simulink model "s_b4a4x1kf"  (R2018a)
settings: Solver=VariableStepDiscrete  StartTime=0.0  StopTime=1  RelTol=1e-3
undefined symbols (not defined in the file): fft_stages, n_bits_ants, n_bits_xengs
libraries: xbsIndex_r4 x22055, xbsReplacements_r4 x30, casper_library_misc x29, casper_library_scopes x15, xps_library x4
(part 72 of 227)

== system s_b4a4x1kf/sys1/vacc_tvg0/ins_vector ==
  new_acc_in : Inport
  data_in : Inport  Port=2
  valid_in : Inport  Port=3
  vector : Inport  Port=4
  value : Inport  Port=5
  enable : Inport  Port=6
  misci : Inport  Port=7
  Delay : xbsIndex_r4/Delay  rst=off  infoeditControl=Selection of Reset will increase slice count due to use of real FFs and instead of SRLs  en=off  latency=2  reg_retiming=off  dbl_ovrd=off  block_type=delay
      settings: xl_area=[0, 0, 0, 0, 0, 0, 0]
  Delay1 : xbsIndex_r4/Delay  rst=off  infoeditControl=Selection of Reset will increase slice count due to use of real FFs and instead of SRLs  en=off  latency=2  reg_retiming=off  dbl_ovrd=off  block_type=delay
      settings: xl_area=[0, 0, 0, 0, 0, 0, 0]
  Delay2 : xbsIndex_r4/Delay  rst=off  infoeditControl=Selection of Reset will increase slice count due to use of real FFs and instead of SRLs  en=off  latency=2  reg_retiming=off  dbl_ovrd=off  block_type=delay
      settings: xl_area=[0, 0, 0, 0, 0, 0, 0]
  Delay3 : xbsIndex_r4/Delay  rst=off  infoeditControl=Selection of Reset will increase slice count due to use of real FFs and instead of SRLs  en=off  latency=3  reg_retiming=on  dbl_ovrd=off  block_type=delay
      settings: xl_area=[0, 0, 0, 0, 0, 0, 0]
  Delay4 : xbsIndex_r4/Delay  rst=off  infoeditControl=Selection of Reset will increase slice count due to use of real FFs and instead of SRLs  en=off  latency=1  reg_retiming=on  dbl_ovrd=off  block_type=delay
      settings: xl_area=[0, 0, 0, 0, 0, 0, 0]
  Delay5 : xbsIndex_r4/Delay  rst=off  infoeditControl=Selection of Reset will increase slice count due to use of real FFs and instead of SRLs  en=off  latency=3  reg_retiming=on  dbl_ovrd=off  block_type=delay
      settings: xl_area=[0, 0, 0, 0, 0, 0, 0]
  Gateway Out{1..6} (6 alike) : xbsIndex_r4/Gateway Out  inherit_from_input=off  hdl_port=off  rows=1  columns=1  UseAsDAC=off  DACChannel='1'  interface=None  automatic_assignment=on  address_offset=hex2dec('00')  intf_name=''  intf_description=''  timing_constraint=None  locs_specified=off  LOCs={}  io_standard={}  block_type=gatewayout
      settings: infoedit="Gateway out block.  Converts Xilinx fixed point inputs into ouputs of type Simulink integer, double, or fixed point.<P><P>Hardware notes:  In hardware these blocks become top level output ports or are discarded, depending on how they are configured."  xl_area=[0, 0, 0, 0, 0, 0, 0]  block_version=10.1.3
  Logical : xbsIndex_r4/Logical  logical_function=AND  inputs=2  en=off  latency=0  precision=Full  arith_type=Unsigned  n_bits=8  bin_pt=2  align_bp=on  dbl_ovrd=off  block_type=logical
      settings: xl_area=[0, 0, 0, 0, 0, 0, 0]
  Mux : xbsIndex_r4/Mux  inputs=2  en=off  latency=1  precision=Full  arith_type="Signed  (2's comp)"  n_bits=8  bin_pt=2  quantization=Truncate  overflow=Wrap  dbl_ovrd=off  block_type=mux
      settings: xl_area=[0, 0, 0, 0, 0, 0, 0]
  Relational : xbsIndex_r4/Relational  mode=a=b  op_type=Bool  en=off  latency=1  dbl_ovrd=off  block_type=relational
      settings: xl_area=[0, 0, 0, 0, 0, 0, 0]  block_version=10.1.3
  Scope2 : Scope  NumInputPorts=6
  tot_cntr : xbsIndex_r4/Counter  cnt_type=Count Limited  cnt_to=num_vectors-1  operation=Up  start_count=0  cnt_by_val=1  arith_type=Unsigned  n_bits=ceil(log2(num_vectors-1))  bin_pt=0  load_pin=off  rst=on  en=on  explicit_period=on  period=1  use_behavioral_HDL=off  implementation=Fabric  use_rpm=on  dbl_ovrd=off  block_type=counter
      settings: xl_area=[0, 0, 0, 0, 0, 0, 0]
  new_acc_out : Outport
  data : Outport  Port=2
  valid_out : Outport  Port=3
  misco : Outport  Port=4
  wires:
  enable/1 -> Logical/1
  Gateway Out5/1 -> Scope2/3
  Gateway Out4/1 -> Scope2/2
  Gateway Out6/1 -> Scope2/1
  Gateway Out1/1 -> Scope2/4
  valid_in/1 -> Delay4/1
  Mux/1 -> data/1, Gateway Out6/1
  tot_cntr/1 -> Gateway Out2/1, Relational/1
  vector/1 -> Relational/2
  data_in/1 -> Delay1/1
  value/1 -> Delay2/1
  Delay/1 -> valid_out/1, Gateway Out4/1
  Logical/1 -> Mux/1, Gateway Out3/1
  Relational/1 -> Logical/2
  Gateway Out2/1 -> Scope2/5
  Delay1/1 -> Mux/2
  Delay3/1 -> new_acc_out/1
  new_acc_in/1 -> Delay3/1, tot_cntr/1, Gateway Out1/1
  Delay4/1 -> tot_cntr/2, Delay/1, Gateway Out5/1
  Delay2/1 -> Mux/3
  Gateway Out3/1 -> Scope2/6
  misci/1 -> Delay5/1
  Delay5/1 -> misco/1

== system s_b4a4x1kf/sys1/vacc_tvg0/n_per_group ==
  sim_1 : Inport
  convert1_1 : DataTypeConversion  OutDataTypeStr=fixdt('ufix32_En0')  LockScale=on
  convert2_1 : DataTypeConversion  OutDataTypeStr=fixdt('ufix32_En0')  ConvertRealWorld=Stored Integer (SI)  LockScale=on
  gain_1 : Gain
  io_delay : xbsIndex_r4/Delay  rst=off  infoeditControl=Selection of Reset will increase slice count due to use of real FFs and instead of SRLs  en=off  latency=0  reg_retiming=on  dbl_ovrd=off  block_type=delay
  reint1 : xbsIndex_r4/Reinterpret  force_arith_type=on  arith_type=Unsigned  force_bin_pt=on  bin_pt=0  block_type=reinterpret
  s_b4a4x1kf_sys1_vacc_tvg0_n_per_group_user_data_out : xbsIndex_r4/Gateway In  gui_display_data_type=Fixed-point  arith_type=Unsigned  n_bits=32  bin_pt=0  preci_type=Single  exp_width=8  frac_width=24  rows=1  columns=1  quantization="Round  (unbiased: +/- Inf)"  overflow=Saturate  period=1  UseAsADC=off  ADCChannel='1'  interface=None  automatic_assignment=on  address_offset=hex2dec('00')  intf_name=''  intf_description=''  default_value=0  timing_constraint=None  locs_specified=off  LOCs={}  io_standard={}  inherit_from_input=off  hdl_port=on  dbl_ovrd=off  block_type=gatewayin
  slice_reg : xbsIndex_r4/Slice  nbits=32  boolean_output=off  mode=Lower Bit Location + Width  bit1=0  base1=MSB of Input  bit0=0  base0=LSB of Input  dbl_ovrd=off  block_type=slice
  in_reg : Outport
  wires:
  s_b4a4x1kf_sys1_vacc_tvg0_n_per_group_user_data_out/1 -> io_delay/1
  sim_1/1 -> convert1_1/1
  convert1_1/1 -> convert2_1/1
  convert2_1/1 -> gain_1/1
  gain_1/1 -> s_b4a4x1kf_sys1_vacc_tvg0_n_per_group_user_data_out/1
  io_delay/1 -> slice_reg/1
  slice_reg/1 -> reint1/1
  reint1/1 -> in_reg/1

== system s_b4a4x1kf/sys1/vacc_tvg0/n_pulses ==
  sim_1 : Inport
  convert1_1 : DataTypeConversion  OutDataTypeStr=fixdt('ufix32_En0')  LockScale=on
  convert2_1 : DataTypeConversion  OutDataTypeStr=fixdt('ufix32_En0')  ConvertRealWorld=Stored Integer (SI)  LockScale=on
  gain_1 : Gain
  io_delay : xbsIndex_r4/Delay  rst=off  infoeditControl=Selection of Reset will increase slice count due to use of real FFs and instead of SRLs  en=off  latency=0  reg_retiming=on  dbl_ovrd=off  block_type=delay
  reint1 : xbsIndex_r4/Reinterpret  force_arith_type=on  arith_type=Unsigned  force_bin_pt=on  bin_pt=0  block_type=reinterpret
  s_b4a4x1kf_sys1_vacc_tvg0_n_pulses_user_data_out : xbsIndex_r4/Gateway In  gui_display_data_type=Fixed-point  arith_type=Unsigned  n_bits=32  bin_pt=0  preci_type=Single  exp_width=8  frac_width=24  rows=1  columns=1  quantization="Round  (unbiased: +/- Inf)"  overflow=Saturate  period=1  UseAsADC=off  ADCChannel='1'  interface=None  automatic_assignment=on  address_offset=hex2dec('00')  intf_name=''  intf_description=''  default_value=0  timing_constraint=None  locs_specified=off  LOCs={}  io_standard={}  inherit_from_input=off  hdl_port=on  dbl_ovrd=off  block_type=gatewayin
  slice_reg : xbsIndex_r4/Slice  nbits=32  boolean_output=off  mode=Lower Bit Location + Width  bit1=0  base1=MSB of Input  bit0=0  base0=LSB of Input  dbl_ovrd=off  block_type=slice
  in_reg : Outport
  wires:
  s_b4a4x1kf_sys1_vacc_tvg0_n_pulses_user_data_out/1 -> io_delay/1
  sim_1/1 -> convert1_1/1
  convert1_1/1 -> convert2_1/1
  convert2_1/1 -> gain_1/1
  gain_1/1 -> s_b4a4x1kf_sys1_vacc_tvg0_n_pulses_user_data_out/1
  io_delay/1 -> slice_reg/1
  slice_reg/1 -> reint1/1
  reint1/1 -> in_reg/1

== system s_b4a4x1kf/sys1/vacc_tvg0/pipeline1 ==
  d : Inport
  Register0 : xbsIndex_r4/Register  init=0  rst=off  en=off  dbl_ovrd=off  block_type=register
      settings: block_version=11.4
  Register1 : xbsIndex_r4/Register  init=0  rst=off  en=off  dbl_ovrd=off  block_type=register
      settings: block_version=11.4
  Register2 : xbsIndex_r4/Register  init=0  rst=off  en=off  dbl_ovrd=off  block_type=register
      settings: block_version=11.4
  q : Outport
  wires:
  Register0/1 -> Register1/1
  Register1/1 -> Register2/1
  d/1 -> Register0/1
  Register2/1 -> q/1

== system s_b4a4x1kf/sys1/vacc_tvg0/pipeline2 ==
  d : Inport
  Register0 : xbsIndex_r4/Register  init=0  rst=off  en=off  dbl_ovrd=off  block_type=register
      settings: block_version=11.4
  Register1 : xbsIndex_r4/Register  init=0  rst=off  en=off  dbl_ovrd=off  block_type=register
      settings: block_version=11.4
  Register2 : xbsIndex_r4/Register  init=0  rst=off  en=off  dbl_ovrd=off  block_type=register
      settings: block_version=11.4
  q : Outport
  wires:
  Register0/1 -> Register1/1
  Register1/1 -> Register2/1
  d/1 -> Register0/1
  Register2/1 -> q/1

== system s_b4a4x1kf/sys1/vacc_tvg0/pipeline3 ==
  d : Inport
  Register0 : xbsIndex_r4/Register  init=0  rst=off  en=off  dbl_ovrd=off  block_type=register
      settings: block_version=11.4
  Register1 : xbsIndex_r4/Register  init=0  rst=off  en=off  dbl_ovrd=off  block_type=register
      settings: block_version=11.4
  Register2 : xbsIndex_r4/Register  init=0  rst=off  en=off  dbl_ovrd=off  block_type=register
      settings: block_version=11.4
  q : Outport
  wires:
  Register0/1 -> Register1/1
  Register1/1 -> Register2/1
  d/1 -> Register0/1
  Register2/1 -> q/1

== system s_b4a4x1kf/sys1/vacc_tvg0/pipeline4 ==
  d : Inport
  Register0 : xbsIndex_r4/Register  init=0  rst=off  en=off  dbl_ovrd=off  block_type=register
      settings: block_version=11.4
  Register1 : xbsIndex_r4/Register  init=0  rst=off  en=off  dbl_ovrd=off  block_type=register
      settings: block_version=11.4
  Register2 : xbsIndex_r4/Register  init=0  rst=off  en=off  dbl_ovrd=off  block_type=register
      settings: block_version=11.4
  q : Outport
  wires:
  Register0/1 -> Register1/1
  Register1/1 -> Register2/1
  d/1 -> Register0/1
  Register2/1 -> q/1

== system s_b4a4x1kf/sys1/vacc_tvg0/pipeline7 ==
  d : Inport
  Register0 : xbsIndex_r4/Register  init=0  rst=off  en=off  dbl_ovrd=off  block_type=register
      settings: block_version=11.4
  Register1 : xbsIndex_r4/Register  init=0  rst=off  en=off  dbl_ovrd=off  block_type=register
      settings: block_version=11.4
  Register2 : xbsIndex_r4/Register  init=0  rst=off  en=off  dbl_ovrd=off  block_type=register
      settings: block_version=11.4
  q : Outport
  wires:
  Register0/1 -> Register1/1
  Register1/1 -> Register2/1
  d/1 -> Register0/1
  Register2/1 -> q/1

== system s_b4a4x1kf/sys1/vacc_tvg0/ts_offset ==
  sim_1 : Inport
  convert1_1 : DataTypeConversion  OutDataTypeStr=fixdt('ufix32_En0')  LockScale=on
  convert2_1 : DataTypeConversion  OutDataTypeStr=fixdt('ufix32_En0')  ConvertRealWorld=Stored Integer (SI)  LockScale=on
  gain_1 : Gain
  io_delay : xbsIndex_r4/Delay  rst=off  infoeditControl=Selection of Reset will increase slice count due to use of real FFs and instead of SRLs  en=off  latency=0  reg_retiming=on  dbl_ovrd=off  block_type=delay
  reint1 : xbsIndex_r4/Reinterpret  force_arith_type=on  arith_type=Unsigned  force_bin_pt=on  bin_pt=0  block_type=reinterpret
  s_b4a4x1kf_sys1_vacc_tvg0_ts_offset_user_data_out : xbsIndex_r4/Gateway In  gui_display_data_type=Fixed-point  arith_type=Unsigned  n_bits=32  bin_pt=0  preci_type=Single  exp_width=8  frac_width=24  rows=1  columns=1  quantization="Round  (unbiased: +/- Inf)"  overflow=Saturate  period=1  UseAsADC=off  ADCChannel='1'  interface=None  automatic_assignment=on  address_offset=hex2dec('00')  intf_name=''  intf_description=''  default_value=0  timing_constraint=None  locs_specified=off  LOCs={}  io_standard={}  inherit_from_input=off  hdl_port=on  dbl_ovrd=off  block_type=gatewayin
  slice_reg : xbsIndex_r4/Slice  nbits=32  boolean_output=off  mode=Lower Bit Location + Width  bit1=0  base1=MSB of Input  bit0=0  base0=LSB of Input  dbl_ovrd=off  block_type=slice
  in_reg : Outport
  wires:
  s_b4a4x1kf_sys1_vacc_tvg0_ts_offset_user_data_out/1 -> io_delay/1
  sim_1/1 -> convert1_1/1
  convert1_1/1 -> convert2_1/1
  convert2_1/1 -> gain_1/1
  gain_1/1 -> s_b4a4x1kf_sys1_vacc_tvg0_ts_offset_user_data_out/1
  io_delay/1 -> slice_reg/1
  slice_reg/1 -> reint1/1
  reint1/1 -> in_reg/1

== system s_b4a4x1kf/sys1/vacc_tvg0/write ==
  sim_1 : Inport
  convert1_1 : DataTypeConversion  OutDataTypeStr=fixdt('ufix32_En0')  LockScale=on
  convert2_1 : DataTypeConversion  OutDataTypeStr=fixdt('ufix32_En0')  ConvertRealWorld=Stored Integer (SI)  LockScale=on
  gain_1 : Gain
  io_delay : xbsIndex_r4/Delay  rst=off  infoeditControl=Selection of Reset will increase slice count due to use of real FFs and instead of SRLs  en=off  latency=0  reg_retiming=on  dbl_ovrd=off  block_type=delay
  reint1 : xbsIndex_r4/Reinterpret  force_arith_type=on  arith_type=Unsigned  force_bin_pt=on  bin_pt=0  block_type=reinterpret
  s_b4a4x1kf_sys1_vacc_tvg0_write_user_data_out : xbsIndex_r4/Gateway In  gui_display_data_type=Fixed-point  arith_type=Unsigned  n_bits=32  bin_pt=0  preci_type=Single  exp_width=8  frac_width=24  rows=1  columns=1  quantization="Round  (unbiased: +/- Inf)"  overflow=Saturate  period=1  UseAsADC=off  ADCChannel='1'  interface=None  automatic_assignment=on  address_offset=hex2dec('00')  intf_name=''  intf_description=''  default_value=0  timing_constraint=None  locs_specified=off  LOCs={}  io_standard={}  inherit_from_input=off  hdl_port=on  dbl_ovrd=off  block_type=gatewayin
  slice_reg : xbsIndex_r4/Slice  nbits=32  boolean_output=off  mode=Lower Bit Location + Width  bit1=0  base1=MSB of Input  bit0=0  base0=LSB of Input  dbl_ovrd=off  block_type=slice
  in_reg : Outport
  wires:
  s_b4a4x1kf_sys1_vacc_tvg0_write_user_data_out/1 -> io_delay/1
  sim_1/1 -> convert1_1/1
  convert1_1/1 -> convert2_1/1
  convert2_1/1 -> gain_1/1
  gain_1/1 -> s_b4a4x1kf_sys1_vacc_tvg0_write_user_data_out/1
  io_delay/1 -> slice_reg/1
  slice_reg/1 -> reint1/1
  reint1/1 -> in_reg/1

== system s_b4a4x1kf/sys1/xeng/auto_tap ==
  a_del : Inport
  a_ndel : Inport  Port=2
  a_loop : Inport  Port=3
  acc_in : Inport  Port=4
  valid_in : Inport  Port=5
  sync_in : Inport  Port=6
  delay : Subsystem  mask(delay_bram){DelayLen=510, bram_latency=7, use_dsp48=off, async=off}
      mask prompts: DelayLen "Delay By:"; bram_latency "BRAM Latency"; use_dsp48 "Use DSP48"; async "asynchronous operation"
      mask help: A delay block that uses BRAM for its storage.
      mask init:
      | delay_bram_init(gcb, ...
      |     'DelayLen', DelayLen, ...
      |     'bram_latency', bram_latency, ...
      |     'use_dsp48', use_dsp48, ...
      |     'async', async);
      mask Help: eval('xlWeb(''http://casper.berkeley.edu/wiki/Delay_bram'')')
  dual_pol_cmac : Subsystem  mask{acc_len=256, n_bits_in=8, bin_pt_in=7, mult_latency=4, add_latency=3, multiplier_implementation=embedded multiplier core}
      mask prompts: acc_len "Number of accumulations"; n_bits_in "Number of bits in"; bin_pt_in "Binary point in"; mult_latency "Multiplier latency"; add_latency "Adder latency"; multiplier_implementation "Multiplier implementation"
      mask init: same as s_b4a4x1kf/sys0/xeng/auto_tap/dual_pol_cmac
      mask TypeOptions multiplier_implementation: behavioral HDL | standard core | embedded multiplier core
  sync_delay : Subsystem  mask(sync_delay){DelayLen=267}
      mask prompts: DelayLen "Delay Length:"
      mask help: Delay an infrequent boolean pulse by the specified number of clocks.
      mask init:
      | BitWidth = max(2, ceil(log2(DelayLen+1)));
      | UseCounter = 1;
      | if DelayLen == 0,
      | 	UseCounter = 0;
      | end
      mask Help: eval('xlWeb(''http://casper.berkeley.edu/wiki/Sync_delay'')')
      mask Display: fprintf('Z^-%d', DelayLen)
  a_del_out : Outport
  a_ndel_out : Outport  Port=2
  a_end_out : Outport  Port=3
  acc_out : Outport  Port=4
  valid_out : Outport  Port=5
  rst_out : Outport  Port=6
  sync_out : Outport  Port=7
  wires:
  sync_delay/1(Out) -> sync_out/1
  delay/1(dout) -> a_end_out/1
  a_loop/1 -> delay/1(din)
  a_ndel/1 -> a_ndel_out/1, dual_pol_cmac/2(a2)
  valid_in/1 -> dual_pol_cmac/5(valid_in)
  dual_pol_cmac/2(valid_out) -> valid_out/1
  acc_in/1 -> dual_pol_cmac/3(acc_in)
  dual_pol_cmac/1(acc_out) -> acc_out/1
  a_del/1 -> a_del_out/1, dual_pol_cmac/1(a1)
  sync_in/1 -> rst_out/1, dual_pol_cmac/4(sync), sync_delay/1(In)

== system s_b4a4x1kf/sys1/xeng/baseline_tap1 ==
  a_del : Inport
  a_ndel : Inport  Port=2
  a_end : Inport  Port=3
  acc_in : Inport  Port=4
  valid_in : Inport  Port=5
  rst : Inport  Port=6
  sync1 : Inport  Port=7
  Constant : xbsIndex_r4/Constant  const=ant_sep * acc_len  gui_display_data_type=Fixed-point  arith_type=Unsigned  n_bits=ant_bits + bit_growth  bin_pt=0  preci_type=Single  exp_width=8  frac_width=24  explicit_period=on  period=1  equ=P=C  opselect=C  inp2=PCIN>>17  opr=+  inp1=P  carry=CIN  dbl_ovrd=off  block_type=constant
      settings: block_version=9.1.01
  Convert : xbsIndex_r4/Convert  gui_display_data_type=Fixed-point  arith_type=Unsigned  n_bits=1  bin_pt=0  float_type=Single  exp_bits=8  fraction_bits=24  quantization=Truncate  overflow=Wrap  en=off  latency=0  pipeline=off  dbl_ovrd=off  block_type=convert
      settings: xl_area=[0, 0, 0, 0, 0, 0, 0]
  Counter : xbsIndex_r4/Counter  cnt_type=Count Limited  cnt_to=n_ants * acc_len - 1  operation=Up  start_count=0  cnt_by_val=1  arith_type=Unsigned  n_bits=ant_bits + bit_growth  bin_pt=0  load_pin=off  rst=on  en=off  explicit_period=off  period=1  use_behavioral_HDL=off  implementation=Fabric  use_rpm=on  dbl_ovrd=off  block_type=counter
      settings: xl_area=[0, 0, 0, 0, 0, 0, 0]  block_version=9.1.01
  Delay{1,3,7..8} (4 alike) : xbsIndex_r4/Delay  rst=off  infoeditControl=Selection of Reset will increase slice count due to use of real FFs and instead of SRLs  en=off  latency=1  reg_retiming=on  dbl_ovrd=off  block_type=delay
      settings: xl_area=[0, 0, 0, 0, 0, 0, 0]  block_version=9.1.01
  Mux : xbsIndex_r4/Mux  inputs=2  en=off  latency=1  precision=Full  arith_type="Signed  (2's comp)"  n_bits=8  bin_pt=2  quantization=Truncate  overflow=Wrap  dbl_ovrd=off  block_type=mux
      settings: xl_area=[0, 0, 0, 0, 0, 0, 0]  block_version=9.1.01
  Relational : xbsIndex_r4/Relational  mode=a<b  op_type=Bool  en=off  latency=0  dbl_ovrd=off  block_type=relational
      settings: xl_area=[0, 0, 0, 0, 0, 0, 0]  block_version=9.1.01
  delay : Subsystem  mask(delay_bram){DelayLen=acc_len, bram_latency=bram_latency, use_dsp48=off, async=off}
      mask prompts: DelayLen "Delay By:"; bram_latency "BRAM Latency"; use_dsp48 "Use DSP48"; async "asynchronous operation"
      mask help: A delay block that uses BRAM for its storage.
      mask init:
      | delay_bram_init(gcb, ...
      |     'DelayLen', DelayLen, ...
      |     'bram_latency', bram_latency, ...
      |     'use_dsp48', use_dsp48, ...
      |     'async', async);
      mask Help: eval('xlWeb(''http://casper.berkeley.edu/wiki/Delay_bram'')')
  dual_pol_cmac : Subsystem  mask{acc_len=256, n_bits_in=8, bin_pt_in=7, mult_latency=4, add_latency=3, multiplier_implementation=embedded multiplier core}
      mask prompts: acc_len "Number of accumulations"; n_bits_in "Number of bits in"; bin_pt_in "Binary point in"; mult_latency "Multiplier latency"; add_latency "Adder latency"; multiplier_implementation "Multiplier implementation"
      mask init: same as s_b4a4x1kf/sys0/xeng/auto_tap/dual_pol_cmac
      mask TypeOptions multiplier_implementation: behavioral HDL | standard core | embedded multiplier core
  a_del_out : Outport
  a_ndel_out : Outport  Port=2
  a_end_out : Outport  Port=3
  acc_out : Outport  Port=4
  valid_out : Outport  Port=5
  rst_out : Outport  Port=6
  sync_out : Outport  Port=7
  wires:
  delay/1(dout) -> Delay3/1
  Mux/1 -> dual_pol_cmac/2(a2)
  Counter/1 -> Relational/1
  Constant/1 -> Relational/2
  Relational/1 -> Convert/1
  Convert/1 -> Mux/1
  rst/1 -> Delay1/1, Counter/1
  a_del/1 -> delay/1(din)
  dual_pol_cmac/1(acc_out) -> acc_out/1
  acc_in/1 -> dual_pol_cmac/3(acc_in)
  dual_pol_cmac/2(valid_out) -> valid_out/1
  valid_in/1 -> dual_pol_cmac/5(valid_in)
  a_ndel/1 -> Mux/2, Delay7/1
  a_end/1 -> Mux/3, Delay8/1
  Delay3/1 -> a_del_out/1, dual_pol_cmac/1(a1)
  Delay7/1 -> a_ndel_out/1
  Delay8/1 -> a_end_out/1
  Delay1/1 -> rst_out/1, dual_pol_cmac/4(sync)
  sync1/1 -> sync_out/1

== system s_b4a4x1kf/sys1/xeng/baseline_tap2 ==
  a_del : Inport
  a_ndel : Inport  Port=2
  a_end : Inport  Port=3
  acc_in : Inport  Port=4
  valid_in : Inport  Port=5
  rst : Inport  Port=6
  sync1 : Inport  Port=7
  Constant : xbsIndex_r4/Constant  const=ant_sep * acc_len  gui_display_data_type=Fixed-point  arith_type=Unsigned  n_bits=ant_bits + bit_growth  bin_pt=0  preci_type=Single  exp_width=8  frac_width=24  explicit_period=on  period=1  equ=P=C  opselect=C  inp2=PCIN>>17  opr=+  inp1=P  carry=CIN  dbl_ovrd=off  block_type=constant
      settings: block_version=9.1.01
  Convert : xbsIndex_r4/Convert  gui_display_data_type=Fixed-point  arith_type=Unsigned  n_bits=1  bin_pt=0  float_type=Single  exp_bits=8  fraction_bits=24  quantization=Truncate  overflow=Wrap  en=off  latency=0  pipeline=off  dbl_ovrd=off  block_type=convert
      settings: xl_area=[0, 0, 0, 0, 0, 0, 0]
  Counter : xbsIndex_r4/Counter  cnt_type=Count Limited  cnt_to=n_ants * acc_len - 1  operation=Up  start_count=0  cnt_by_val=1  arith_type=Unsigned  n_bits=ant_bits + bit_growth  bin_pt=0  load_pin=off  rst=on  en=off  explicit_period=off  period=1  use_behavioral_HDL=off  implementation=Fabric  use_rpm=on  dbl_ovrd=off  block_type=counter
      settings: xl_area=[0, 0, 0, 0, 0, 0, 0]  block_version=9.1.01
  Delay{1,3,7..8} (4 alike) : xbsIndex_r4/Delay  rst=off  infoeditControl=Selection of Reset will increase slice count due to use of real FFs and instead of SRLs  en=off  latency=1  reg_retiming=on  dbl_ovrd=off  block_type=delay
      settings: xl_area=[0, 0, 0, 0, 0, 0, 0]  block_version=9.1.01
  Mux : xbsIndex_r4/Mux  inputs=2  en=off  latency=1  precision=Full  arith_type="Signed  (2's comp)"  n_bits=8  bin_pt=2  quantization=Truncate  overflow=Wrap  dbl_ovrd=off  block_type=mux
      settings: xl_area=[0, 0, 0, 0, 0, 0, 0]  block_version=9.1.01
  Relational : xbsIndex_r4/Relational  mode=a<b  op_type=Bool  en=off  latency=0  dbl_ovrd=off  block_type=relational
      settings: xl_area=[0, 0, 0, 0, 0, 0, 0]  block_version=9.1.01
  delay : Subsystem  mask(delay_bram){DelayLen=acc_len, bram_latency=bram_latency, use_dsp48=off, async=off}
      mask prompts: DelayLen "Delay By:"; bram_latency "BRAM Latency"; use_dsp48 "Use DSP48"; async "asynchronous operation"
      mask help: A delay block that uses BRAM for its storage.
      mask init:
      | delay_bram_init(gcb, ...
      |     'DelayLen', DelayLen, ...
      |     'bram_latency', bram_latency, ...
      |     'use_dsp48', use_dsp48, ...
      |     'async', async);
      mask Help: eval('xlWeb(''http://casper.berkeley.edu/wiki/Delay_bram'')')
  dual_pol_cmac : Subsystem  mask{acc_len=256, n_bits_in=8, bin_pt_in=7, mult_latency=4, add_latency=3, multiplier_implementation=embedded multiplier core}
      mask prompts: acc_len "Number of accumulations"; n_bits_in "Number of bits in"; bin_pt_in "Binary point in"; mult_latency "Multiplier latency"; add_latency "Adder latency"; multiplier_implementation "Multiplier implementation"
      mask init: same as s_b4a4x1kf/sys0/xeng/auto_tap/dual_pol_cmac
      mask TypeOptions multiplier_implementation: behavioral HDL | standard core | embedded multiplier core
  a_del_out : Outport
  a_ndel_out : Outport  Port=2
  a_end_out : Outport  Port=3
  acc_out : Outport  Port=4
  valid_out : Outport  Port=5
  rst_out : Outport  Port=6
  sync_out : Outport  Port=7
  wires:
  delay/1(dout) -> Delay3/1
  Mux/1 -> dual_pol_cmac/2(a2)
  Counter/1 -> Relational/1
  Constant/1 -> Relational/2
  Relational/1 -> Convert/1
  Convert/1 -> Mux/1
  rst/1 -> Delay1/1, Counter/1
  a_del/1 -> delay/1(din)
  dual_pol_cmac/1(acc_out) -> acc_out/1
  acc_in/1 -> dual_pol_cmac/3(acc_in)
  dual_pol_cmac/2(valid_out) -> valid_out/1
  valid_in/1 -> dual_pol_cmac/5(valid_in)
  a_ndel/1 -> Mux/2, Delay7/1
  a_end/1 -> Mux/3, Delay8/1
  Delay3/1 -> a_del_out/1, dual_pol_cmac/1(a1)
  Delay7/1 -> a_ndel_out/1
  Delay8/1 -> a_end_out/1
  Delay1/1 -> rst_out/1, dual_pol_cmac/4(sync)
  sync1/1 -> sync_out/1

== system s_b4a4x1kf/sys1/xeng/sample_and_hold1 ==
  sync : Inport
  in : Inport  Port=2
  Constant3 : xbsIndex_r4/Constant  const=period-1  gui_display_data_type=Fixed-point  arith_type=Unsigned  n_bits=ceil(log2(period))  bin_pt=0  preci_type=Single  exp_width=8  frac_width=24  explicit_period=on  period=1  equ=P=C  opselect=C  inp2=PCIN>>17  opr=+  inp1=P  carry=CIN  dbl_ovrd=off  block_type=constant
  Counter4 : xbsIndex_r4/Counter  cnt_type=Free Running  cnt_to=Inf  operation=Up  start_count=0  cnt_by_val=1  arith_type=Unsigned  n_bits=ceil(log2(period))  bin_pt=0  load_pin=off  rst=on  en=off  explicit_period=on  period=1  use_behavioral_HDL=off  implementation=Fabric  use_rpm=on  dbl_ovrd=off  block_type=counter
      settings: xl_area=[0, 0, 0, 0, 0, 0, 0]
  Delay10 : xbsIndex_r4/Delay  rst=off  infoeditControl=Selection of Reset will increase slice count due to use of real FFs and instead of SRLs  en=off  latency=1  reg_retiming=on  dbl_ovrd=off  block_type=delay
      settings: xl_area=[0, 0, 0, 0, 0, 0, 0]
  Logical : xbsIndex_r4/Logical  logical_function=OR  inputs=2  en=off  latency=0  precision=Full  arith_type=Unsigned  n_bits=16  bin_pt=0  align_bp=on  dbl_ovrd=off  block_type=logical
  Register : xbsIndex_r4/Register  init=0  rst=off  en=on  dbl_ovrd=off  block_type=register
  Relational : xbsIndex_r4/Relational  mode=a>=b  op_type=Bool  en=off  latency=0  dbl_ovrd=off  block_type=relational
      settings: xl_area=[0, 0, 0, 0, 0, 0, 0]  block_version=10.1.3
  out : Outport
  wires:
  Relational/1 -> Logical/1
  Constant3/1 -> Relational/2
  Counter4/1 -> Relational/1
  Logical/1 -> Counter4/1, Delay10/1
  sync/1 -> Logical/2
  Register/1 -> out/1
  in/1 -> Register/1
  Delay10/1 -> Register/2

== system s_b4a4x1kf/sys1/xeng/sample_and_hold2 ==
  sync : Inport
  in : Inport  Port=2
  Constant3 : xbsIndex_r4/Constant  const=period-1  gui_display_data_type=Fixed-point  arith_type=Unsigned  n_bits=ceil(log2(period))  bin_pt=0  preci_type=Single  exp_width=8  frac_width=24  explicit_period=on  period=1  equ=P=C  opselect=C  inp2=PCIN>>17  opr=+  inp1=P  carry=CIN  dbl_ovrd=off  block_type=constant
  Counter4 : xbsIndex_r4/Counter  cnt_type=Free Running  cnt_to=Inf  operation=Up  start_count=0  cnt_by_val=1  arith_type=Unsigned  n_bits=ceil(log2(period))  bin_pt=0  load_pin=off  rst=on  en=off  explicit_period=on  period=1  use_behavioral_HDL=off  implementation=Fabric  use_rpm=on  dbl_ovrd=off  block_type=counter
      settings: xl_area=[0, 0, 0, 0, 0, 0, 0]
  Delay10 : xbsIndex_r4/Delay  rst=off  infoeditControl=Selection of Reset will increase slice count due to use of real FFs and instead of SRLs  en=off  latency=1  reg_retiming=on  dbl_ovrd=off  block_type=delay
      settings: xl_area=[0, 0, 0, 0, 0, 0, 0]
  Logical : xbsIndex_r4/Logical  logical_function=OR  inputs=2  en=off  latency=0  precision=Full  arith_type=Unsigned  n_bits=16  bin_pt=0  align_bp=on  dbl_ovrd=off  block_type=logical
  Register : xbsIndex_r4/Register  init=0  rst=off  en=on  dbl_ovrd=off  block_type=register
  Relational : xbsIndex_r4/Relational  mode=a>=b  op_type=Bool  en=off  latency=0  dbl_ovrd=off  block_type=relational
      settings: xl_area=[0, 0, 0, 0, 0, 0, 0]  block_version=10.1.3
  out : Outport
  wires:
  Relational/1 -> Logical/1
  Constant3/1 -> Relational/2
  Counter4/1 -> Relational/1
  Logical/1 -> Counter4/1, Delay10/1
  sync/1 -> Logical/2
  Register/1 -> out/1
  in/1 -> Register/1
  Delay10/1 -> Register/2

== system s_b4a4x1kf/sys1/xeng/sample_and_hold3 ==
  sync : Inport
  in : Inport  Port=2
  Constant3 : xbsIndex_r4/Constant  const=period-1  gui_display_data_type=Fixed-point  arith_type=Unsigned  n_bits=ceil(log2(period))  bin_pt=0  preci_type=Single  exp_width=8  frac_width=24  explicit_period=on  period=1  equ=P=C  opselect=C  inp2=PCIN>>17  opr=+  inp1=P  carry=CIN  dbl_ovrd=off  block_type=constant
  Counter4 : xbsIndex_r4/Counter  cnt_type=Free Running  cnt_to=Inf  operation=Up  start_count=0  cnt_by_val=1  arith_type=Unsigned  n_bits=ceil(log2(period))  bin_pt=0  load_pin=off  rst=on  en=off  explicit_period=on  period=1  use_behavioral_HDL=off  implementation=Fabric  use_rpm=on  dbl_ovrd=off  block_type=counter
      settings: xl_area=[0, 0, 0, 0, 0, 0, 0]
  Delay10 : xbsIndex_r4/Delay  rst=off  infoeditControl=Selection of Reset will increase slice count due to use of real FFs and instead of SRLs  en=off  latency=1  reg_retiming=on  dbl_ovrd=off  block_type=delay
      settings: xl_area=[0, 0, 0, 0, 0, 0, 0]
  Logical : xbsIndex_r4/Logical  logical_function=OR  inputs=2  en=off  latency=0  precision=Full  arith_type=Unsigned  n_bits=16  bin_pt=0  align_bp=on  dbl_ovrd=off  block_type=logical
  Register : xbsIndex_r4/Register  init=0  rst=off  en=on  dbl_ovrd=off  block_type=register
  Relational : xbsIndex_r4/Relational  mode=a>=b  op_type=Bool  en=off  latency=0  dbl_ovrd=off  block_type=relational
      settings: xl_area=[0, 0, 0, 0, 0, 0, 0]  block_version=10.1.3
  out : Outport
  wires:
  Relational/1 -> Logical/1
  Constant3/1 -> Relational/2
  Counter4/1 -> Relational/1
  Logical/1 -> Counter4/1, Delay10/1
  sync/1 -> Logical/2
  Register/1 -> out/1
  in/1 -> Register/1
  Delay10/1 -> Register/2

== system s_b4a4x1kf/sys1/xeng/window_delay ==
  in : Inport
  Gateway Out{2..3,55..56} (4 alike) : xbsIndex_r4/Gateway Out  inherit_from_input=off  hdl_port=on  rows=1  columns=1  UseAsDAC=off  DACChannel='1'  interface=None  automatic_assignment=on  address_offset=hex2dec('00')  intf_name=''  intf_description=''  timing_constraint=None  locs_specified=off  LOCs={}  io_standard={}  block_type=gatewayout
      settings: infoedit="Gateway out block.  Converts Xilinx fixed point inputs into ouputs of type Simulink integer, double, or fixed point.<P><P>Hardware notes:  In hardware these blocks become top level output ports or are discarded, depending on how they are configured."  xl_area=[0, 0, 0, 0, 0, 0, 0]  block_version=9.2.01
  Register : xbsIndex_r4/Register  init=0  rst=on  en=on  dbl_ovrd=off  block_type=register
      settings: xl_area=[0, 0, 0, 0, 0, 0, 0]  block_version=9.2.01
  Scope1 : Scope  NumInputPorts=4
  negedge : Subsystem  mask(edge_detect){edge=Falling, polarity=Active High, x_in=[0 0.08 0.08 0.16 0.16 0.24 0.24 0.32 0.32 0.4], y_in=[1  1 -1 -1 -1 -1 -1 -1 -1 -1], x_out=[0.6 0.68 0.68 0.76 0.76 0.84 0.84 0.92 0.92 1], y_out=[-1 -1  1  1 -1 -1 -1 -1 -1 -1]}
      mask prompts: edge "Edge Type"; polarity "Output Polarity"; x_in "Input X Positions"; y_in "Input Y Positions"; x_out "Output X Positions"; y_out "Output Y Positions"
      mask help: Output is active for one-cycle after each edge of the specified type (i.e. rising, falling or both).
      mask init: same as s_b4a4x1kf/edge_detect
      settings: AttributesFormatString=|
      | falling edges
      | active high
      mask Help: Output is active for one-cycle after each edge of the specified type (i.e. rising, falling, or both).  Latency is zero.
      mask TypeOptions edge: Rising | Falling | Both
      mask TypeOptions polarity: Active High | Active Low
      mask Display:
      | plot(x_in_num,0.5+y_in_num*0.2);
      | plot(x_out_num,0.5+y_out_num*0.2);
  posedge3 : Subsystem  mask(edge_detect){edge=Rising, polarity=Active High, x_in=[0 0.08 0.08 0.16 0.16 0.24 0.24 0.32 0.32 0.4], y_in=[-1 -1  1  1  1  1  1  1  1  1], x_out=[0.6 0.68 0.68 0.76 0.76 0.84 0.84 0.92 0.92 1], y_out=[-1 -1  1  1 -1 -1 -1 -1 -1 -1]}
      mask prompts: edge "Edge Type"; polarity "Output Polarity"; x_in "Input X Positions"; y_in "Input Y Positions"; x_out "Output X Positions"; y_out "Output Y Positions"
      mask help: Output is active for one-cycle after each edge of the specified type (i.e. rising, falling or both).
      mask init: same as s_b4a4x1kf/edge_detect
      settings: AttributesFormatString=|
      | rising edges
      | active high
      mask Help: Output is active for one-cycle after each edge of the specified type (i.e. rising, falling, or both).  Latency is zero.
      mask TypeOptions edge: Rising | Falling | Both
      mask TypeOptions polarity: Active High | Active Low
      mask Display:
      | plot(x_in_num,0.5+y_in_num*0.2);
      | plot(x_out_num,0.5+y_out_num*0.2);
  sync_delay : Subsystem  mask(sync_delay){DelayLen=delay-1}
      mask prompts: DelayLen "Delay Length:"
      mask help: Delay an infrequent boolean pulse by the specified number of clocks.
      mask init:
      | BitWidth = max(2, ceil(log2(DelayLen+1)));
      | UseCounter = 1;
      | if DelayLen == 0,
      | 	UseCounter = 0;
      | end
      mask Help: eval('xlWeb(''http://casper.berkeley.edu/wiki/Sync_delay'')')
      mask Display: fprintf('Z^-%d', DelayLen)
  sync_delay1 : Subsystem  mask(sync_delay){DelayLen=delay-1}
      mask prompts: DelayLen "Delay Length:"
      mask help: Delay an infrequent boolean pulse by the specified number of clocks.
      mask init:
      | BitWidth = max(2, ceil(log2(DelayLen+1)));
      | UseCounter = 1;
      | if DelayLen == 0,
      | 	UseCounter = 0;
      | end
      mask Help: eval('xlWeb(''http://casper.berkeley.edu/wiki/Sync_delay'')')
      mask Display: fprintf('Z^-%d', DelayLen)
  out : Outport
  wires:
  Register/1 -> Gateway Out3/1, out/1
  sync_delay1/1(Out) -> Gateway Out2/1, Register/2
  sync_delay/1(Out) -> Gateway Out56/1, Register/3, Register/1
  negedge/1(out) -> sync_delay1/1(In)
  posedge3/1(out) -> sync_delay/1(In)
  in/1 -> Gateway Out55/1, posedge3/1(in), negedge/1(in)
  Gateway Out3/1 -> Scope1/4
  Gateway Out2/1 -> Scope1/3
  Gateway Out56/1 -> Scope1/2
  Gateway Out55/1 -> Scope1/1

== system s_b4a4x1kf/sys1/xeng/xeng_descramble_4ant ==
  note: This bit of logic
      | ensures that we only send out
      | a sync if one was received
      | (and then align it with the start of a read)
  note: x_cast is necessary to correct for BRAM
      | readout order
  acc : Inport
  valid : Inport  Port=2
  sync : Inport  Port=3
  win_valid : Inport  Port=4
  Constant2 : xbsIndex_r4/Constant  const=0  gui_display_data_type=Fixed-point  arith_type=Boolean  n_bits=elements_bits + 1  bin_pt=0  preci_type=Single  exp_width=8  frac_width=24  explicit_period=on  period=1  equ=P=C  opselect=C  inp2=PCIN>>17  opr=+  inp1=P  carry=CIN  dbl_ovrd=off  block_type=constant
      settings: block_version=9.2.01
  Constant3 : xbsIndex_r4/Constant  const=0  gui_display_data_type=Fixed-point  arith_type=Unsigned  n_bits=n_bits_in/demux_factor  bin_pt=0  preci_type=Single  exp_width=8  frac_width=24  explicit_period=on  period=1  equ=P=C  opselect=C  inp2=PCIN>>17  opr=+  inp1=P  carry=CIN  dbl_ovrd=off  block_type=constant
      settings: block_version=9.2.01
  Delay{1..6} (6 alike) : xbsIndex_r4/Delay  rst=off  infoeditControl=Selection of Reset will increase slice count due to use of real FFs and instead of SRLs  en=off  latency=2  reg_retiming=off  dbl_ovrd=off  block_type=delay
      Delay1 settings: infoedit=Hardware notes: A delay line is a chain, each link of which is an SRL16 or SRL32 followed by a flip-flop.  xl_area=[0, 0, 0, 0, 0, 0, 0]  block_version=9.2.01
      Delay2 settings: infoedit=Hardware notes: A delay line is a chain, each link of which is an SRL16 or SRL32 followed by a flip-flop.  xl_area=[0, 0, 0, 0, 0, 0, 0]  block_version=9.2.01
      Delay3 settings: infoedit=Hardware notes: A delay line is a chain, each link of which is an SRL16 or SRL32 followed by a flip-flop.  xl_area=[0, 0, 0, 0, 0, 0, 0]  block_version=9.2.01
      Delay4 settings: infoedit=Hardware notes: A delay line is a chain, each link of which is an SRL16 or SRL32 followed by a flip-flop.  xl_area=[0, 0, 0, 0, 0, 0, 0]  block_version=9.2.01
      Delay5 settings: xl_area=[0, 0, 0, 0, 0, 0, 0]  block_version=9.2.01
      Delay6 settings: xl_area=[0, 0, 0, 0, 0, 0, 0]  block_version=9.2.01
  Dual Port RAM : xbsIndex_r4/Dual Port RAM  depth=(num_elements+1)*demux_factor  initVector=[1:36*8]  distributed_mem=Block RAM  init_a=0  init_b=0  rst_a=off  rst_b=off  en_a=off  en_b=off  latency=2  write_mode_A=No Read On Write  write_mode_B=No Read On Write  optimize=Area  dbl_ovrd=off  block_type=dpram
      settings: xl_area=[0, 0, 0, 0, 0, 0, 0]  block_version=9.2.01
  Gateway Out{1..11,17,19..20} (14 alike) : xbsIndex_r4/Gateway Out  inherit_from_input=off  hdl_port=off  rows=1  columns=1  UseAsDAC=off  DACChannel='1'  interface=None  automatic_assignment=on  address_offset=hex2dec('00')  intf_name=''  intf_description=''  timing_constraint=None  locs_specified=off  LOCs={}  io_standard={}  block_type=gatewayout
      settings: infoedit="Gateway out block.  Converts Xilinx fixed point inputs into ouputs of type Simulink integer, double, or fixed point.<P><P>Hardware notes:  In hardware these blocks become top level output ports or are discarded, depending on how they are configured."  xl_area=[0, 0, 0, 0, 0, 0, 0]  block_version=10.1.3
  Logical : xbsIndex_r4/Logical  logical_function=AND  inputs=2  en=off  latency=2  precision=Full  arith_type=Unsigned  n_bits=16  bin_pt=0  align_bp=on  dbl_ovrd=off  block_type=logical
  Register : xbsIndex_r4/Register  init=0  rst=on  en=on  dbl_ovrd=off  block_type=register
  Scope1 : Scope  NumInputPorts=8
  Scope6 : Scope  NumInputPorts=6
  Terminator1 : Terminator
  read_ctrl : Subsystem
  write_ctrl : Subsystem
  x_cast : Subsystem  mask{n_bits_in=n_bits_xeng_out, n_bits_out=n_bits_in/8, fix_pnt_pos=(n_bits-1)*2, demux_factor=demux_factor}
      mask prompts: n_bits_in "Number of bits (input)"; n_bits_out "Number of bits (output)"; fix_pnt_pos "Fixed point position"; demux_factor "Demux Factor"
      mask init: same as s_b4a4x1kf/sys0/x_cast
      settings: AttributesFormatString=25 -> 32, demux 1.
  acc_out : Outport
  valid_out : Outport  Port=2
  sync_out : Outport  Port=3
  wires:
  Gateway Out11/1 -> Scope1/8
  valid/1 -> write_ctrl/3(xeng_valid), Delay6/1
  sync/1 -> write_ctrl/1(sync), [sync_in]
  write_ctrl/2(write_addr) -> Gateway Out11/1, Dual Port RAM/4
  read_ctrl/1(read_addr) -> Dual Port RAM/1, Delay2/1, Gateway Out9/1
  Dual Port RAM/1 -> Gateway Out1/1, acc_out/1
  Delay1/1 -> Gateway Out2/1, valid_out/1
  Constant2/1 -> Dual Port RAM/3
  write_ctrl/4(enable) -> Gateway Out10/1, Dual Port RAM/6, Delay3/1
  Constant3/1 -> Dual Port RAM/2
  write_ctrl/3(data_out) -> x_cast/1(in)
  acc/1 -> write_ctrl/2(data_in)
  Dual Port RAM/2 -> Terminator1/1
  Gateway Out20/1 -> Scope6/3
  Gateway Out19/1 -> Scope6/2
  Gateway Out17/1 -> Scope6/1
  Gateway Out1/1 -> Scope6/4
  Gateway Out2/1 -> Scope6/5
  Gateway Out3/1 -> Scope6/6
  Gateway Out8/1 -> Scope1/3
  Gateway Out6/1 -> Scope1/2
  Gateway Out5/1 -> Scope1/1
  Gateway Out4/1 -> Scope1/4
  Gateway Out7/1 -> Scope1/5
  Gateway Out9/1 -> Scope1/6
  Gateway Out10/1 -> Scope1/7
  Delay2/1 -> Gateway Out20/1
  Delay3/1 -> Gateway Out19/1
  Delay4/1 -> Gateway Out17/1
  Logical/1 -> Gateway Out3/1, sync_out/1
  Register/1 -> Logical/2
  win_valid/1 -> write_ctrl/4(window_valid), Delay5/1
  write_ctrl/1(start_readout) -> [start_read]
  [start_read] -> read_ctrl/1(start)
  [start_read] -> Logical/1
  [start_read] -> Register/2
  [start_read] -> Gateway Out4/1
  read_ctrl/2(enable) -> [valid_out]
  [valid_out] -> Delay1/1
  [valid_out] -> Gateway Out7/1
  [sync_in] -> Gateway Out5/1
  [sync_in] -> Register/1
  [sync_in] -> Register/3
  Delay5/1 -> Gateway Out8/1
  Delay6/1 -> Gateway Out6/1
  x_cast/1(out) -> Dual Port RAM/5, Delay4/1

== system s_b4a4x1kf/sys1/xeng_pack_out/edge_detect ==
  in : Inport
  Delay : xbsIndex_r4/Delay  rst=off  infoeditControl=Selection of Reset will increase slice count due to use of real FFs and instead of SRLs  en=off  latency=1  reg_retiming=on  dbl_ovrd=off  block_type=delay
      settings: xl_area=[0, 0, 0, 0, 0, 0, 0]
  Inverter : xbsIndex_r4/Inverter  en=off  latency=0  dbl_ovrd=off  block_type=inv
      settings: xl_area=[0, 0, 0, 0, 0, 0, 0]
  edge_op : xbsIndex_r4/Logical  logical_function=NOR  inputs=2  en=off  latency=0  precision=Full  arith_type=Unsigned  n_bits=8  bin_pt=2  align_bp=on  dbl_ovrd=off  block_type=logical
      settings: xl_area=[0, 0, 0, 0, 0, 0, 0]
  out : Outport
  wires:
  Inverter/1 -> edge_op/1
  edge_op/1 -> out/1
  in/1 -> Inverter/1, Delay/1
  Delay/1 -> edge_op/2

== system s_b4a4x1kf/sys1/xeng_pack_out/edge_detect1 ==
  in : Inport
  Delay : xbsIndex_r4/Delay  rst=off  infoeditControl=Selection of Reset will increase slice count due to use of real FFs and instead of SRLs  en=off  latency=1  reg_retiming=on  dbl_ovrd=off  block_type=delay
      settings: xl_area=[0, 0, 0, 0, 0, 0, 0]
  Inverter : xbsIndex_r4/Inverter  en=off  latency=0  dbl_ovrd=off  block_type=inv
      settings: xl_area=[0, 0, 0, 0, 0, 0, 0]
  edge_op : xbsIndex_r4/Logical  logical_function=NOR  inputs=2  en=off  latency=0  precision=Full  arith_type=Unsigned  n_bits=8  bin_pt=2  align_bp=on  dbl_ovrd=off  block_type=logical
      settings: xl_area=[0, 0, 0, 0, 0, 0, 0]
  out : Outport
  wires:
  Delay/1 -> edge_op/2
  in/1 -> Delay/1, Inverter/1
  edge_op/1 -> out/1
  Inverter/1 -> edge_op/1

== system s_b4a4x1kf/sys1/xeng_pack_out/edge_detect2 ==
  in : Inport
  Delay : xbsIndex_r4/Delay  rst=off  infoeditControl=Selection of Reset will increase slice count due to use of real FFs and instead of SRLs  en=off  latency=1  reg_retiming=on  dbl_ovrd=off  block_type=delay
      settings: xl_area=[0, 0, 0, 0, 0, 0, 0]
  Inverter : xbsIndex_r4/Inverter  en=off  latency=0  dbl_ovrd=off  block_type=inv
      settings: xl_area=[0, 0, 0, 0, 0, 0, 0]
  edge_op : xbsIndex_r4/Logical  logical_function=NOR  inputs=2  en=off  latency=0  precision=Full  arith_type=Unsigned  n_bits=8  bin_pt=2  align_bp=on  dbl_ovrd=off  block_type=logical
      settings: xl_area=[0, 0, 0, 0, 0, 0, 0]
  out : Outport
  wires:
  Inverter/1 -> edge_op/1
  edge_op/1 -> out/1
  in/1 -> Inverter/1, Delay/1
  Delay/1 -> edge_op/2

== system s_b4a4x1kf/sys1/xeng_pack_out/edge_detect3 ==
  in : Inport
  Delay : xbsIndex_r4/Delay  rst=off  infoeditControl=Selection of Reset will increase slice count due to use of real FFs and instead of SRLs  en=off  latency=1  reg_retiming=on  dbl_ovrd=off  block_type=delay
      settings: xl_area=[0, 0, 0, 0, 0, 0, 0]
  Inverter : xbsIndex_r4/Inverter  en=off  latency=0  dbl_ovrd=off  block_type=inv
      settings: xl_area=[0, 0, 0, 0, 0, 0, 0]
  edge_op : xbsIndex_r4/Logical  logical_function=NOR  inputs=2  en=off  latency=0  precision=Full  arith_type=Unsigned  n_bits=8  bin_pt=2  align_bp=on  dbl_ovrd=off  block_type=logical
      settings: xl_area=[0, 0, 0, 0, 0, 0, 0]
  out : Outport
  wires:
  Delay/1 -> edge_op/2
  in/1 -> Delay/1, Inverter/1
  edge_op/1 -> out/1
  Inverter/1 -> edge_op/1

== system s_b4a4x1kf/sys1/xeng_pack_out/edge_detect7 ==
  in : Inport
  Delay : xbsIndex_r4/Delay  rst=off  infoeditControl=Selection of Reset will increase slice count due to use of real FFs and instead of SRLs  en=off  latency=1  reg_retiming=on  dbl_ovrd=off  block_type=delay
      settings: xl_area=[0, 0, 0, 0, 0, 0, 0]
  Inverter : xbsIndex_r4/Inverter  en=off  latency=0  dbl_ovrd=off  block_type=inv
      settings: xl_area=[0, 0, 0, 0, 0, 0, 0]
  edge_op : xbsIndex_r4/Logical  logical_function=NOR  inputs=2  en=off  latency=0  precision=Full  arith_type=Unsigned  n_bits=8  bin_pt=2  align_bp=on  dbl_ovrd=off  block_type=logical
      settings: xl_area=[0, 0, 0, 0, 0, 0, 0]
  out : Outport
  wires:
  Delay/1 -> edge_op/2
  in/1 -> Delay/1, Inverter/1
  edge_op/1 -> out/1
  Inverter/1 -> edge_op/1
